simulink model "arducopter"  (R2021a)
settings: Solver=FixedStepAuto  StartTime=0.0  StopTime=simIn.param.timeEnd  FixedStep=simIn.param.dt  RelTol=1e-3
undefined symbols (not defined in the file or in its folder): DiscIntNeverNeededParam, sim, simIn
libraries: simulink x35, slident x4, vrlib x1
(part 4 of 9)

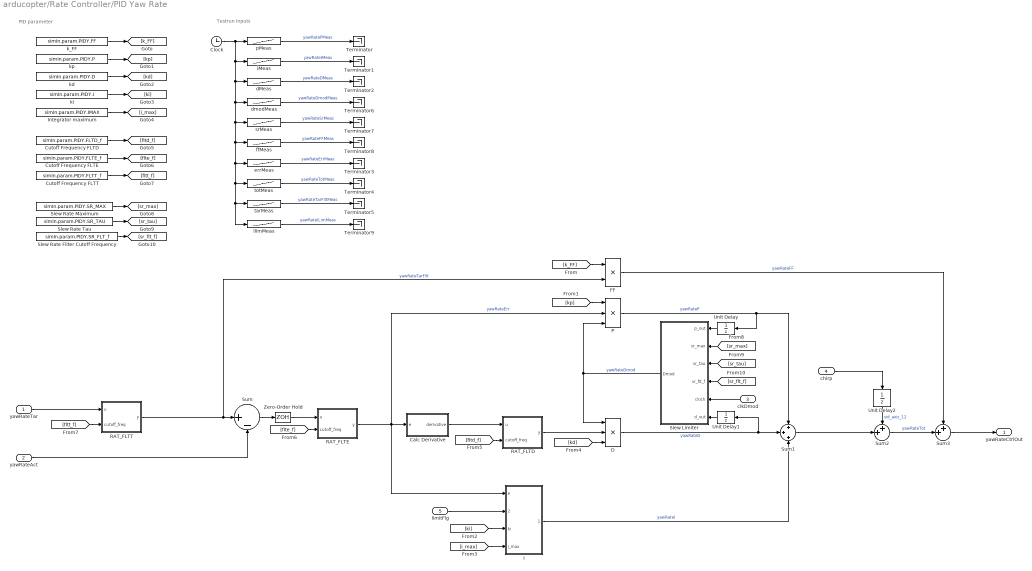
== system arducopter/Rate Controller/PID Yaw Rate ==
  note: PID parameter
  note: Testrun inputs
  yawRateTar : Inport
  yawRateAct : Inport  Port=2
  clkDmod : Inport  Port=3
  chirp : Inport  Port=4
  limitFlg : Inport  Port=5
  Calc Derivative : Subsystem
  Clock : Clock
  Cutoff Frequency FLTD : Constant  Value=simIn.param.PIDY.FLTD_f
  Cutoff Frequency FLTE : Constant  Value=simIn.param.PIDY.FLTE_f
  Cutoff Frequency FLTT : Constant  Value=simIn.param.PIDY.FLTT_f
  D : Product  Inputs=3
  FF : Product
  I : Subsystem
  Integrator maximum : Constant  Value=simIn.param.PIDY.IMAX
  P : Product  Inputs=3
  RAT_FLTD : Subsystem  TreatAsAtomicUnit=on  SystemSampleTime=simIn.param.dt
  RAT_FLTE : Subsystem  TreatAsAtomicUnit=on  SystemSampleTime=simIn.param.dt
  RAT_FLTT : Subsystem  TreatAsAtomicUnit=on  SystemSampleTime=simIn.param.dt
  Slew Limiter : Subsystem
  Slew Rate Filter Cutoff Frequency : Constant  Value=simIn.param.PIDY.SR_FLT_f
  Slew Rate Maximum : Constant  Value=simIn.param.PIDY.SR_MAX
  Slew Rate Tau : Constant  Value=simIn.param.PIDY.SR_TAU
  Sum : Sum  Inputs=|+-
  Sum1 : Sum  Inputs=+|+|+
  Sum2 : Sum  Inputs=++|
  Sum3 : Sum  Inputs=++|  OutDataTypeStr=single
  Terminator{,1..9} (10 alike) : Terminator
  Unit Delay : UnitDelay  InitialCondition=simIn.init.PIDY.P  SampleTime=-1  HasFrameUpgradeWarning=on
  Unit Delay1 : UnitDelay  InitialCondition=simIn.init.PIDY.D  SampleTime=-1  HasFrameUpgradeWarning=on
  Unit Delay2 : UnitDelay  SampleTime=-1  HasFrameUpgradeWarning=on
  Zero-Order Hold : ZeroOrderHold  SampleTime=-1
  dMeas : Lookup_n-D  NumberOfTableDimensions=1  BreakpointsForDimension1=simIn.signals.PIDY.Time  Table=simIn.signals.PIDY.D  InternalRulePriority=Speed  RndMeth=Simplest  InputSameDT=on
  dmodMeas : Lookup_n-D  NumberOfTableDimensions=1  BreakpointsForDimension1=simIn.signals.PIDY.Time  Table=simIn.signals.PIDY.DMod  InternalRulePriority=Speed  RndMeth=Simplest  InputSameDT=on
  errMeas : Lookup_n-D  NumberOfTableDimensions=1  BreakpointsForDimension1=simIn.signals.PIDY.Time  Table=simIn.signals.PIDY.Err  InternalRulePriority=Speed  RndMeth=Simplest  InputSameDT=on
  ffMeas : Lookup_n-D  NumberOfTableDimensions=1  BreakpointsForDimension1=simIn.signals.PIDY.Time  Table=simIn.signals.PIDY.FF  InternalRulePriority=Speed  RndMeth=Simplest  InputSameDT=on
  iMeas : Lookup_n-D  NumberOfTableDimensions=1  BreakpointsForDimension1=simIn.signals.PIDY.Time  Table=simIn.signals.PIDY.I  InternalRulePriority=Speed  RndMeth=Simplest  InputSameDT=on
  ilimMeas : Lookup_n-D  NumberOfTableDimensions=1  BreakpointsForDimension1=simIn.signals.PIDY.Time  Table=simIn.signals.PIDY.ILimit  InternalRulePriority=Speed  RndMeth=Simplest  InputSameDT=on
  k_FF : Constant  Value=simIn.param.PIDY.FF
  kd : Constant  Value=simIn.param.PIDY.D
  ki : Constant  Value=simIn.param.PIDY.I
  kp : Constant  Value=simIn.param.PIDY.P
  pMeas : Lookup_n-D  NumberOfTableDimensions=1  BreakpointsForDimension1=simIn.signals.PIDY.Time  Table=simIn.signals.PIDY.P  InternalRulePriority=Speed  RndMeth=Simplest  InputSameDT=on
  srMeas : Lookup_n-D  NumberOfTableDimensions=1  BreakpointsForDimension1=simIn.signals.PIDY.Time  Table=simIn.signals.PIDY.SRate  InternalRulePriority=Speed  RndMeth=Simplest  InputSameDT=on
  tarMeas : Lookup_n-D  NumberOfTableDimensions=1  BreakpointsForDimension1=simIn.signals.PIDY.Time  Table=simIn.signals.PIDY.Tar  InternalRulePriority=Speed  RndMeth=Simplest  InputSameDT=on
  totMeas : Lookup_n-D  NumberOfTableDimensions=1  BreakpointsForDimension1=simIn.signals.RATE.Time  Table=simIn.signals.RATE.YOut  InternalRulePriority=Speed  RndMeth=Simplest  InputSameDT=on
  yawRateCtrlOut : Outport
  wires:
  RAT_FLTD/1(y) -> D/2
  Sum1/1 -> Sum2/2
  RAT_FLTE/1(y) -> P/2, Calc Derivative/1(e), I/1(e)  "yawRateErr"
  limitFlg/1 -> I/2(limit_flg)
  P/1 -> Unit Delay/1, Sum1/1  "yawRateP"
  Calc Derivative/1(derivative) -> RAT_FLTD/1(u)
  Sum/1 -> Zero-Order Hold/1
  D/1 -> Unit Delay1/1, Sum1/2  "yawRateD"
  I/1(integrator) -> Sum1/3  "yawRateI"
  FF/1 -> Sum3/1  "yawRateFF"
  Sum2/1 -> Sum3/2  "yawRateTot"
  Sum3/1 -> yawRateCtrlOut/1
  RAT_FLTT/1(y) -> FF/2, Sum/1  "yawRateTarFilt"
  yawRateTar/1 -> RAT_FLTT/1(u)
  yawRateAct/1 -> Sum/2
  Zero-Order Hold/1 -> RAT_FLTE/1(u)
  k_FF/1 -> [k_FF]
  kp/1 -> [kp]
  kd/1 -> [kd]
  ki/1 -> [ki]
  Integrator maximum/1 -> [i_max]
  Cutoff Frequency FLTD/1 -> [fltd_f]
  Cutoff Frequency FLTE/1 -> [flte_f]
  Cutoff Frequency FLTT/1 -> [fltt_f]
  [k_FF] -> FF/1
  [kp] -> P/1
  [ki] -> I/3(ki)
  [i_max] -> I/4(i_max)
  [kd] -> D/3
  [fltd_f] -> RAT_FLTD/2(cutoff_freq)
  [flte_f] -> RAT_FLTE/2(cutoff_freq)
  [fltt_f] -> RAT_FLTT/2(cutoff_freq)
  pMeas/1 -> Terminator/1  "yawRatePMeas"
  iMeas/1 -> Terminator1/1  "yawRateIMeas"
  dMeas/1 -> Terminator2/1  "yawRateDMeas"
  totMeas/1 -> Terminator4/1  "yawRateTotMeas"
  tarMeas/1 -> Terminator5/1  "yawRateTarFiltMeas"
  errMeas/1 -> Terminator3/1  "yawRateErrMeas"
  Unit Delay2/1 -> Sum2/1  "sid_axis_12"
  Slew Rate Filter Cutoff Frequency/1 -> [sr_flt_f]
  Slew Rate Maximum/1 -> [sr_max]
  Slew Rate Tau/1 -> [sr_tau]
  dmodMeas/1 -> Terminator6/1  "yawRateDmodMeas"
  srMeas/1 -> Terminator7/1  "yawRateSrMeas"
  ffMeas/1 -> Terminator8/1  "yawRateFFMeas"
  Slew Limiter/1(Dmod) -> D/1, P/3  "yawRateDmod"
  Unit Delay/1 -> Slew Limiter/1(p_out)
  Unit Delay1/1 -> Slew Limiter/6(d_out)
  [sr_max] -> Slew Limiter/2(sr_max)
  [sr_tau] -> Slew Limiter/3(sr_tau)
  [sr_flt_f] -> Slew Limiter/4(sr_flt_f)
  ilimMeas/1 -> Terminator9/1  "yawRateILimMeas"
  clkDmod/1 -> Slew Limiter/5(clock)
  chirp/1 -> Unit Delay2/1
  Clock/1 -> ilimMeas/1, tarMeas/1, totMeas/1, errMeas/1, ffMeas/1, srMeas/1, dmodMeas/1, dMeas/1, iMeas/1, pMeas/1

== system arducopter/Throttle/Input Handler ==
  note: Input Handler
      | Determines source of the inputs to the subsystem, which can
      | be either the real flight data or simulated data.
  inMeas : Inport
  inSim : Inport  Port=2
  thrMan : Inport  Port=3
  Bus Creator : BusCreator  Inputs=9
  Bus Selector : BusSelector  OutputSignals=throttle.thrIn
  Bus Selector1 : BusSelector  OutputSignals=CTUN.thrInMeas,CTUN.angBst,BAT.batRestVoltEst,BAT.batCurr,BAT.batRes,BAT.batVolt,BARO.baroAlt,BARO.baroAirPress,BARO.baroGndTemp
  Switch : Switch  Criteria=u2 > Threshold
  data_in : Outport
  wires:
  inSim/1 -> Bus Selector/1
  inMeas/1 -> Bus Selector1/1
  thrMan/1 -> Switch/2
  Bus Selector/1 -> Switch/3  "<thrIn>"
  Bus Selector1/1 -> Switch/1  "<thrInMeas>"
  Bus Selector1/9 -> Bus Creator/9  "<baroGndTemp>"
  Bus Selector1/8 -> Bus Creator/8  "<baroAirPress>"
  Bus Selector1/7 -> Bus Creator/7  "<baroAlt>"
  Bus Selector1/6 -> Bus Creator/6  "<batVolt>"
  Bus Selector1/5 -> Bus Creator/5  "<batRes>"
  Bus Selector1/4 -> Bus Creator/4  "<batCurr>"
  Bus Selector1/3 -> Bus Creator/3  "<batRestVoltEst>"
  Bus Selector1/2 -> Bus Creator/2  "<angBst>"
  Switch/1 -> Bus Creator/1  "thrTar"
  Bus Creator/1 -> data_in/1

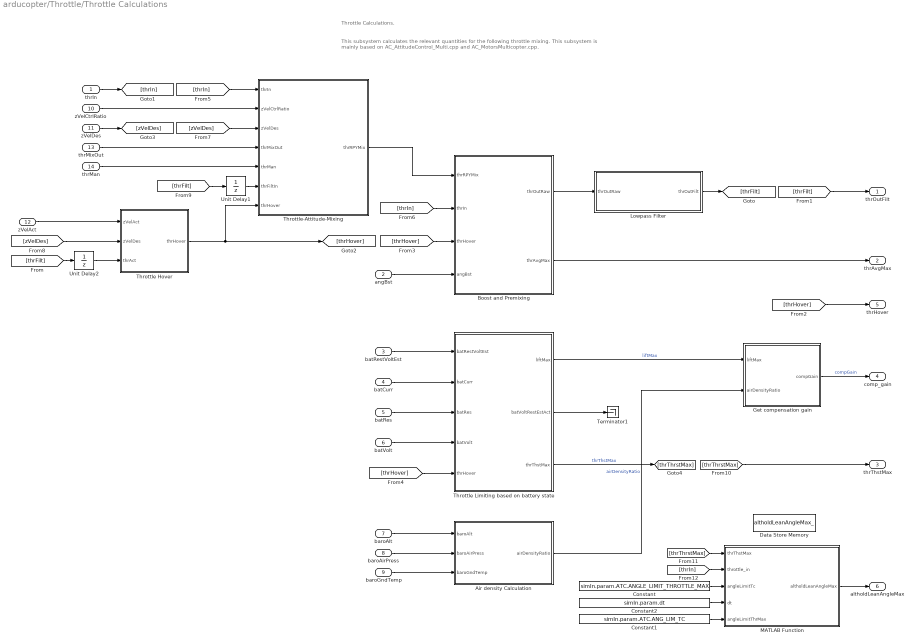
== system arducopter/Throttle/Throttle Calculations ==
  note: Throttle Calculations.
  note: This subsystem calculates the relevant quantities for the following throttle mixing.
      | This subsystem is mainly based on AC_AttitudeControl_Multi.cpp and AC_MotorsMulticopter.cpp.
  thrIn : Inport
  angBst : Inport  Port=2
  batRestVoltEst : Inport  Port=3
  batCurr : Inport  Port=4
  batRes : Inport  Port=5
  batVolt : Inport  Port=6
  baroAlt : Inport  Port=7
  baroAirPress : Inport  Port=8
  baroGndTemp : Inport  Port=9
  zVelCtrlRatio : Inport  Port=10
  zVelDes : Inport  Port=11
  zVelAct : Inport  Port=12
  thrMixOut : Inport  Port=13
  thrMan : Inport  Port=14
  Air density Calculation : Subsystem
  Boost and Premixing : Subsystem  TreatAsAtomicUnit=on  SystemSampleTime=simIn.param.dt
  Constant : Constant  Value=simIn.param.ATC.ANGLE_LIMIT_THROTTLE_MAX
  Constant1 : Constant  Value=simIn.param.ATC.ANG_LIM_TC
  Constant2 : Constant  Value=simIn.param.dt
  Data Store Memory : DataStoreMemory  DataStoreName=altholdLeanAngleMax_  ReadBeforeWriteMsg=warning  WriteAfterWriteMsg=warning  WriteAfterReadMsg=warning  InitialValue=single(0)  ShowAdditionalParam=off  OutDataTypeStr=single
  Get compensation gain : MATLAB Function  TreatAsAtomicUnit=on
  Lowpass Filter : Subsystem
  MATLAB Function : MATLAB Function  TreatAsAtomicUnit=on
  Terminator1 : Terminator
  Throttle Hover : Subsystem  TreatAsAtomicUnit=on  SystemSampleTime=0.1
  Throttle Limiting based on battery state : Subsystem
  Throttle-Attitude-Mixing : Subsystem
  Unit Delay1 : UnitDelay  InitialCondition=simIn.init.CTUN.ThrOut  SampleTime=-1  HasFrameUpgradeWarning=on
  Unit Delay2 : UnitDelay  InitialCondition=simIn.init.CTUN.ThrOut  SampleTime=-1  HasFrameUpgradeWarning=on
  thrOutFilt : Outport
  thrAvgMax : Outport  Port=2
  thrThstMax : Outport  Port=3
  comp_gain : Outport  Port=4
  thrHover : Outport  Port=5
  altholdLeanAngleMax : Outport  Port=6
  wires:
  Throttle Hover/1(thrHover) -> [thrHover], Throttle-Attitude-Mixing/7(thrHover)
  Get compensation gain/1(compGain) -> comp_gain/1  "compGain"
  Throttle Limiting based on battery state/1(liftMax) -> Get compensation gain/1(liftMax)  "liftMax"
  [thrFilt] -> Unit Delay2/1
  Throttle Limiting based on battery state/2(batVoltRestEstAct) -> Terminator1/1
  [thrHover] -> Throttle Limiting based on battery state/5(thrHover)
  Unit Delay2/1 -> Throttle Hover/3(thrAct)
  Throttle Limiting based on battery state/3(thrThstMax) -> [thrThrstMax]  "thrThstMax"
  [thrFilt] -> thrOutFilt/1
  Lowpass Filter/1(thrOutFilt) -> [thrFilt]
  angBst/1 -> Boost and Premixing/4(angBst)
  [thrHover] -> Boost and Premixing/3(thrHover)
  Boost and Premixing/2(thrAvgMax) -> thrAvgMax/1
  batRestVoltEst/1 -> Throttle Limiting based on battery state/1(batRestVoltEst)
  batCurr/1 -> Throttle Limiting based on battery state/2(batCurr)
  batRes/1 -> Throttle Limiting based on battery state/3(batRes)
  batVolt/1 -> Throttle Limiting based on battery state/4(batVolt)
  baroAlt/1 -> Air density Calculation/1(baroAlt)
  baroAirPress/1 -> Air density Calculation/2(baroAirPress)
  baroGndTemp/1 -> Air density Calculation/3(baroGndTemp)
  Boost and Premixing/1(thrOutRaw) -> Lowpass Filter/1(thrOutRaw)
  [thrHover] -> thrHover/1
  [thrIn] -> Boost and Premixing/2(thrIn)
  thrIn/1 -> [thrIn]
  zVelCtrlRatio/1 -> Throttle-Attitude-Mixing/2(zVelCtrlRatio)
  thrMan/1 -> Throttle-Attitude-Mixing/5(thrMan)
  Throttle-Attitude-Mixing/1(thrRPYMix) -> Boost and Premixing/1(thrRPYMix)
  [thrIn] -> Throttle-Attitude-Mixing/1(thrIn)
  zVelDes/1 -> [zVelDes]
  [zVelDes] -> Throttle-Attitude-Mixing/3(zVelDes)
  [zVelDes] -> Throttle Hover/2(zVelDes)
  zVelAct/1 -> Throttle Hover/1(zVelAct)
  Air density Calculation/1(airDensityRatio) -> Get compensation gain/2(airDensityRatio)  "airDensityRatio"
  thrMixOut/1 -> Throttle-Attitude-Mixing/4(thrMixOut)
  [thrFilt] -> Unit Delay1/1
  Unit Delay1/1 -> Throttle-Attitude-Mixing/6(thrFiltIn)
  [thrThrstMax] -> thrThstMax/1
  [thrThrstMax] -> MATLAB Function/1(thrThstMax)
  [thrIn] -> MATLAB Function/2(throttle_in)
  Constant/1 -> MATLAB Function/3(angleLimitTc)
  Constant1/1 -> MATLAB Function/5(angleLimitThrMax)
  Constant2/1 -> MATLAB Function/4(dt)
  MATLAB Function/1(altholdLeanAngleMax) -> altholdLeanAngleMax/1

== system arducopter/Attitude Controller/input_euler_angle_roll_pitch_euler_rate_yaw()/Add feedforward to angVelBody ==
  note: Thrust error angle above which yaw corrections are limited
  angVelBodyFeedforward : Inport
  angVelBodyIn : Inport  Port=2
  thurstErrorAngle : Inport  Port=3
  yawRateAct : Inport  Port=4
  Constant : Constant  Value=simIn.param.ATC.THRUST_ERROR_ANGLE
  MATLAB Function : MATLAB Function  TreatAsAtomicUnit=on
  angVelBody : Outport
  feedforwardScaler : Outport  Port=2
  wires:
  angVelBodyFeedforward/1 -> MATLAB Function/1(angVelBodyFeedforward)
  angVelBodyIn/1 -> MATLAB Function/2(angVelBodyIn)
  thurstErrorAngle/1 -> MATLAB Function/3(thrustErrorAngle)
  yawRateAct/1 -> MATLAB Function/4(yawRateAct)
  MATLAB Function/1(angVelBodyNew) -> angVelBody/1
  Constant/1 -> MATLAB Function/5(maxThrustErrorAngle4YawCorr)
  MATLAB Function/2(feedforwardScaler) -> feedforwardScaler/1

== system arducopter/Attitude Controller/input_euler_angle_roll_pitch_euler_rate_yaw()/Feedforward disabled ==
  note: QuaternionT<T>::from_euler()
      | Computes the quaternion from the given euler angles
  note: This subsystem represents to part of input_euler_angle_roll_pitch_euler_rate_yaw() that is executed, when the feedforward is disabled ( ATC_RATE_FF_ENAB = 0 )
  eulerAngleTar : Inport
  eulerInputDes : Inport  Port=2
  Constant : Constant  Value=0  OutDataTypeStr=single
  Constant1 : Constant  Value=0  OutDataTypeStr=single
  Demux : Demux  Outputs=3
  Gain : Gain  Gain=simIn.param.dt
  MATLAB Function : MATLAB Function  TreatAsAtomicUnit=on
  Selector : Selector  InputPortWidth=3  IndexOptions=Index vector (dialog)  Indices=[3]  OutputSizes=1
  Sum : Sum  Inputs=|++
  eulerRateTar : Outport
  angVelTar : Outport  Port=2
  attitudeTarget : Outport  Port=3
  wires:
  MATLAB Function/1(q) -> attitudeTarget/1  "attitudeTarget"
  Demux/1 -> MATLAB Function/1(roll)
  Demux/2 -> MATLAB Function/2(pitch)
  eulerInputDes/1 -> Demux/1
  Demux/3 -> Gain/1
  Gain/1 -> Sum/1
  Sum/1 -> MATLAB Function/3(yaw)
  eulerAngleTar/1 -> Selector/1
  Constant/1 -> eulerRateTar/1
  Constant1/1 -> angVelTar/1
  Selector/1 -> Sum/2

== system arducopter/Attitude Controller/input_euler_angle_roll_pitch_euler_rate_yaw()/Feedforward enabled ==
  note: euler_rate_to_ang_vel()
      | Converts the target euler rates into a target frame angular velocity vector for feedforward
  note: euler_accel_limit()
      | Translation of acceleration limits eulerAccelMax to the body frame
  note: This subsystem represents to part of input_euler_angle_roll_pitch_euler_rate_yaw() that is executed, when the feedforward is enabled (ATC_RATE_FF_ENAB = 1)
  note: Maximum angular accelerations in earth frame
  note: Input shaping
      | Computes target euler rates based on the error between latest angle target and the desired angle by the pilot, thereby considering acceleration limits.
  note: ang_vel_limit()
      | Ensures that angular velocites do not go over configured rate limits
  note: ang_vel_to_euler_rate()
      | Converts the target body-frame angular velocites into target euler rates
  eulerRateTarIn : Inport
  eulerAngleTar : Inport  Port=2
  eulerInputDes : Inport  Port=3
  Constant : Constant  Value=simIn.param.ATC.ACCEL_R_MAX
  Constant1 : Constant  Value=simIn.param.ATC.ACCEL_P_MAX
  Constant2 : Constant  Value=simIn.param.ATC.ACCEL_Y_MAX
  Constant3 : Constant  Value=simIn.param.ATC.RATE_R_MAX
  Constant4 : Constant  Value=simIn.param.ATC.RATE_P_MAX
  Constant5 : Constant  Value=simIn.param.ATC.RATE_Y_MAX
  Gain : Gain  Gain=pi/180
  Gain1 : Gain  Gain=pi/180
  Gain2 : Gain  Gain=pi/180
  MATLAB Function : MATLAB Function  TreatAsAtomicUnit=on
  MATLAB Function1 : MATLAB Function  TreatAsAtomicUnit=on
  MATLAB Function2 : MATLAB Function  TreatAsAtomicUnit=on
  MATLAB Function3 : MATLAB Function  TreatAsAtomicUnit=on
  Mux : Mux  Inputs=3
  cdeg/ss to rad/ss : Gain  Gain=0.01*pi/180
  input shaping : Subsystem
  eulerRateTarOut : Outport
  angVelTar : Outport  Port=2
  wires:
  [eulerAngleTar] -> MATLAB Function/1(eulerAngleTar), MATLAB Function1/1(eulerAngle), input shaping/1(eulerAngleTar)
  Constant/1 -> Mux/1
  Mux/1 -> cdeg/ss to rad/ss/1
  Constant1/1 -> Mux/2
  Constant2/1 -> Mux/3
  MATLAB Function/1(eulerAccelMaxBF) -> input shaping/4(eulerAccelMax)
  eulerInputDes/1 -> input shaping/2(eulerInputDes)
  eulerRateTarIn/1 -> input shaping/3(eulerRateTarIn)
  input shaping/1(eulerRateTar) -> MATLAB Function1/2(eulerRate)  "eulerRateTar"
  MATLAB Function1/1(angVelTar) -> MATLAB Function2/1(angVelTar)  "angVelTar"
  Gain/1 -> MATLAB Function2/2(angVelRollMax)
  Constant3/1 -> Gain/1
  Constant4/1 -> Gain1/1
  Gain1/1 -> MATLAB Function2/3(angVelPitchMax)
  Gain2/1 -> MATLAB Function2/4(angVelYawMax)
  Constant5/1 -> Gain2/1
  eulerAngleTar/1 -> [eulerAngleTar]  "eulerAngleTar"
  [eulerAngleTar] -> MATLAB Function3/2(eulerAngle)
  MATLAB Function3/1(eulerRate) -> eulerRateTarOut/1
  MATLAB Function2/1(angVelTarLimited) -> [angVelTar]
  [angVelTar] -> MATLAB Function3/1(angVelBf)
  [angVelTar] -> angVelTar/1
  cdeg/ss to rad/ss/1 -> MATLAB Function/2(eulerAccelMaxEF)

== system arducopter/Attitude Controller/input_euler_angle_roll_pitch_euler_rate_yaw()/Update attitudeTarget ==
  note: Normalize attitudeTarget
  note: Use angVelTar to rotate attitudeTarget
  note: Use rotated attitudeTarget, if FF is enabled.
      | Otherwise, use unchanged attitudeTarget
  attitudeTarget : Inport
  angVelTar : Inport  Port=2
  ffEnabled : Inport  Port=3
  MATLAB Function : MATLAB Function  TreatAsAtomicUnit=on
  Rotate target attitude : Subsystem
  Switch : Switch  Criteria=u2 > Threshold
  attitudeTargetUpdate : Outport
  wires:
  MATLAB Function/1(qNorm) -> attitudeTargetUpdate/1
  Switch/1 -> MATLAB Function/1(q)
  ffEnabled/1 -> Switch/2
  attitudeTarget/1 -> Switch/3, Rotate target attitude/1(attitudeTarget)
  angVelTar/1 -> Rotate target attitude/2(angVelTar)
  Rotate target attitude/1(attitudeTargetRot) -> Switch/1

== system arducopter/Attitude Controller/input_euler_angle_roll_pitch_euler_rate_yaw()/reset yaw targets ==
  note: "ahrs.yaw - euler_angle_target.z"
  note: This subsystem resets the yaw target angle and rate, if the throttle is zero, meaning that the copter is landed. The respective function is AC_AttitudeControl::reset_yaw_target_and_rate() , which is called in ModeStabilize::run() when the copter is armed, but throttle is still zero.
  eulerRateTarIn : Inport
  attitudeTargetIn : Inport  Port=2
  eulerAngleAct : Inport  Port=3
  throttle : Inport  Port=4
  Demux : Demux  Outputs=3
  Demux1 : Demux  Outputs=3
  MATLAB Function1 : MATLAB Function  TreatAsAtomicUnit=on
  MATLAB Function5 : MATLAB Function  TreatAsAtomicUnit=on
  MATLAB Function9 : MATLAB Function  TreatAsAtomicUnit=on
  Mux : Mux  Inputs=3
  Mux1 : Mux  Inputs=3
  Subtract : Sum  Inputs=-+
  Switch : Switch  Criteria=u2 > Threshold
  Switch1 : Switch  Criteria=u2 > Threshold
  Terminator{,1..4} (5 alike) : Terminator
  Zero : Constant  Value=0  OutDataTypeStr=single
  Zero1 : Constant  Value=0  OutDataTypeStr=single
  Zero2 : Constant  Value=0  OutDataTypeStr=single
  eulerRateTar : Outport
  attitudeTarget : Outport  Port=2
  wires:
  Switch1/1 -> attitudeTarget/1
  Switch/1 -> eulerRateTar/1
  throttle/1 -> Switch1/2, Switch/2
  eulerRateTarIn/1 -> Demux1/1, Switch/1
  eulerAngleAct/1 -> Demux/1
  MATLAB Function9/1(qRes) -> Switch1/3
  attitudeTargetIn/1 -> Switch1/1, MATLAB Function9/2(q2), MATLAB Function1/1(q)
  MATLAB Function1/3(yaw) -> Subtract/1  "yawAngleTar"
  MATLAB Function1/1(roll) -> Terminator/1
  MATLAB Function1/2(pitch) -> Terminator1/1
  Demux/1 -> Terminator2/1
  Demux/2 -> Terminator3/1
  Demux/3 -> Subtract/2
  Subtract/1 -> Mux/3
  MATLAB Function5/1(q) -> MATLAB Function9/1(q1)  "attitudeTargetUpdate"
  Mux/1 -> MATLAB Function5/1(vec)
  Zero/1 -> Mux/1
  Zero1/1 -> Mux/2
  Mux1/1 -> Switch/3
  Demux1/1 -> Mux1/1
  Demux1/2 -> Mux1/2
  Demux1/3 -> Terminator4/1
  Zero2/1 -> Mux1/3

== system arducopter/Attitude Controller/input_euler_angle_roll_pitch_euler_rate_yaw()/thrust_heading_rotation_angles() ==
  note: Limit yaw error based in maximum acceleration
  note: AC_AttitudeControl::thrust_vector_rotation_angles()
      | Calculation of thrust_angle, thrust_error_angle, attitude_error and thrust_vector_correction
  note: This subsystem contains all the calculations contained in the function AC_AttitudeControl::thrust_heading_rotation_angles() that is called in AC_AttitudeControl::attitude_controller_run_quat()
  attitudeTargetIn : Inport
  attitudeBodyAct : Inport  Port=2
  Yaw error limitation : Subsystem
  thrust_vector_rotation_angles() : Subsystem
  attitudeTarget : Outport
  attitudeError : Outport  Port=2
  thrustErrorAngle : Outport  Port=3
  thrustAngle : Outport  Port=4
  wires:
  attitudeTargetIn/1 -> [attitudeTarget]  "attTar"
  [attitudeBody] -> thrust_vector_rotation_angles()/2(attitudeBodyAct)
  thrust_vector_rotation_angles()/1(attitudeError) -> Yaw error limitation/1(attitudeErrorIn)
  thrust_vector_rotation_angles()/3(thrustErrAngle) -> thrustErrorAngle/1
  thrust_vector_rotation_angles()/2(thrustVecCorrection) -> Yaw error limitation/2(thrustVecCorrection)
  thrust_vector_rotation_angles()/4(thrustAngle) -> thrustAngle/1
  attitudeBodyAct/1 -> [attitudeBody]  "attBody"
  [attitudeBody] -> Yaw error limitation/3(attitudeBody)
  Yaw error limitation/1(atitudeTarget) -> attitudeTarget/1
  Yaw error limitation/2(attitudeError) -> attitudeError/1
  [attitudeTarget] -> thrust_vector_rotation_angles()/1(attitudeTarget)
  [attitudeTarget] -> Yaw error limitation/4(attitudeTarget)

== system arducopter/Attitude Controller/input_euler_angle_roll_pitch_euler_rate_yaw()/update_ang_vel_target_from_att_error() ==
  note: The subsystems either use the square root controller or an easy proportional relation (kp*err) to calculate the target angular velocity
  note: AC_AttitudeControl::update_ang_vel_target_from_att_error()
      | Compute the angular velocity corrections in the body frame from the attitude error.
  attitudeError : Inport
  Calc angular velocity target pitch : Subsystem
  Calc angular velocity target roll : Subsystem
  Calc angular velocity target yaw : Subsystem
  Mux : Mux  Inputs=3
  Selector : Selector  InputPortWidth=3  IndexOptions=Index vector (dialog)  Indices=[1]  OutputSizes=1
  Selector1 : Selector  InputPortWidth=3  IndexOptions=Index vector (dialog)  Indices=[2]  OutputSizes=1
  Selector2 : Selector  InputPortWidth=3  IndexOptions=Index vector (dialog)  Indices=[3]  OutputSizes=1
  angVelBody : Outport
  wires:
  attitudeError/1 -> Selector2/1, Selector/1, Selector1/1
  Mux/1 -> angVelBody/1
  Selector/1 -> Calc angular velocity target roll/1(attitudeErrorRoll)
  Calc angular velocity target roll/1(angVelRoll) -> Mux/1
  Calc angular velocity target yaw/1(angVelYaw) -> Mux/3
  Calc angular velocity target pitch/1(angVelPitch) -> Mux/2
  Selector1/1 -> Calc angular velocity target pitch/1(attitudeErrorPitch)
  Selector2/1 -> Calc angular velocity target yaw/1(attitudeErrorYaw)

== system arducopter/Position Controller/P Position z/Scale Factor Z ==
  note: AP_AHRS::getControlScaleZ()
      | This subsystem calculates a scaling factor for the target of vertical motion quantities based on the EKF type that is being used.
      | Taken from AP_AHRS::getControlScaleZ() in AP_AHRS.cpp. Called in AC_PosControl::update_z_controller().
      | Flying with only DCM lower the gain of the controllers by 4x to cope with high lag.
  ekfType : Inport
  EKF used : Constant  OutDataTypeStr=single
  No EKF : Constant  Value=0.25  OutDataTypeStr=single
  Switch : Switch  Criteria=u2 > Threshold
  scale_z : Outport
  wires:
  ekfType/1 -> Switch/2
  EKF used/1 -> Switch/1
  No EKF/1 -> Switch/3
  Switch/1 -> scale_z/1

== system arducopter/Position Controller/P Position z/Set vertical speed & acceleration limit ==
  note: Calculation of vertical speed and acceleration limits
      | This subsystem corresponds to the function set_correction_speed_accel_z() , in AC_PosControl.cpp,
      | which is called in the ModeLoiter::init() function of mode_loiter.cpp.
      | The intention of this function is to calculate z position error limits, which corresponds to the vertical speed
      | and acceleration limits given by parameters, so that the speed and acceleration limits are still kept after
      | the square root controller was executed without explicitly enforce the limits to the quantities.
  outMin : Inport
  outMax : Inport  Port=2
  DoutMax : Inport  Port=3
  D2OutMax : Inport  Port=4
  kp : Inport  Port=5
  Abs : Abs
  Gain : Gain  Gain=-1
  Inverse Square Root Controller : Subsystem  TreatAsAtomicUnit=on
  Set error limits : MATLAB Function  TreatAsAtomicUnit=on
  errMin : Outport
  errMax : Outport  Port=2
  D1max : Outport  Port=3
  wires:
  Abs/1 -> Gain/1
  Gain/1 -> Set error limits/1(outMin)
  outMax/1 -> Set error limits/2(outMax)
  outMin/1 -> Abs/1
  DoutMax/1 -> Set error limits/3(DoutMax)
  Set error limits/1(errMin) -> errMin/1
  Set error limits/3(D1max) -> D1max/1
  Set error limits/2(errMax) -> errMax/1
  D2OutMax/1 -> Set error limits/4(D2OutMax)
  kp/1 -> Set error limits/5(kp)

== system arducopter/Position Controller/PID Acceleration z/Calc Derivative ==
  e : Inport
  ATC input time constant : Constant  Value=simIn.param.dt
  Divide : Product  Inputs=*/
  Sum : Sum  Inputs=|+-
  Unit Delay : UnitDelay  SampleTime=-1  HasFrameUpgradeWarning=on
  derivative : Outport
  wires:
  e/1 -> Sum/1, Unit Delay/1
  Unit Delay/1 -> Sum/2
  Sum/1 -> Divide/1
  ATC input time constant/1 -> Divide/2
  Divide/1 -> derivative/1

== system arducopter/Position Controller/PID Acceleration z/I ==
  note: Integrator, see AC_PID.cpp, line 230
      | Initialization: set_integrator() in AC_PosControl::init_z_controller()
  e : Inport
  limitFlg : Inport  Port=2
  ki : Inport  Port=3
  i_max : Inport  Port=4
  Constant1 : Constant  Value=simIn.param.dt
  Data Type Conversion1 : DataTypeConversion  OutDataTypeStr=single
  IC1 : InitialCondition  Value=simIn.init.PIDA.I
  Integrator : MATLAB Function  TreatAsAtomicUnit=on
  Unit Delay1 : UnitDelay  InitialCondition=simIn.init.PIDA.I  SampleTime=-1  HasFrameUpgradeWarning=on
  integrator : Outport
  wires:
  e/1 -> Integrator/1(error)
  Integrator/1(integrator_out) -> IC1/1
  [integrator_out] -> integrator/1
  Constant1/1 -> Data Type Conversion1/1
  limitFlg/1 -> Integrator/3(limit_flg)
  [integrator_out] -> Unit Delay1/1
  IC1/1 -> [integrator_out]
  Unit Delay1/1 -> Integrator/2(integrator)
  ki/1 -> Integrator/4(ki)
  i_max/1 -> Integrator/5(i_max)
  Data Type Conversion1/1 -> Integrator/6(dt)

== system arducopter/Position Controller/PID Acceleration z/RAT_FLTD ==
  note: Digital Filter:
      | $y_n = (1 - \alpha)y_{n-1} + x \cdot \alpha$
  note: Alpha Calculation:
      | $\alpha = \frac{\mathrm{d}t}{\mathrm{d}t + 2 \pi f_{\mathrm{Cutoff}}$
  note: See AC_PID.cpp, line 144.
  note: See AP_Math.cpp, line 393.
  u : Inport
  cutoff_freq : Inport  Port=2
  ATC input time constant : Constant  Value=simIn.param.dt
  Add : Sum
  Calculate Alpha : Product  Inputs=*/
  Compare To Zero : simulink/Logic and Bit Operations/Compare To Zero  relop=<=  OutDataTypeStr=boolean
  Compare To Zero1 : simulink/Logic and Bit Operations/Compare To Zero  relop=<=  OutDataTypeStr=boolean
  Constant2 : Constant  OutDataTypeStr=single
  Constant3 : Constant  OutDataTypeStr=single
  Constant4 : Constant  OutDataTypeStr=single
  Data Type Conversion1 : DataTypeConversion  OutDataTypeStr=single
  Divide : Product  Inputs=*/
  Gain : Gain  Gain=2*pi
  IC : InitialCondition  Value=simIn.init.PIDA.DerFilt
  Logical Operator : Logic  Operator=OR  AllPortsSameDT=off  OutDataTypeStr=boolean
  Product : Product
  Product1 : Product
  Subtract1 : Sum  Inputs=+-
  Sum : Sum  Inputs=++|  OutDataTypeStr=single
  Switch : Switch  Criteria=u2 > Threshold
  Unit Delay : UnitDelay  SampleTime=-1  HasFrameUpgradeWarning=on
  y : Outport
  wires:
  Product1/1 -> Sum/2
  Unit Delay/1 -> Product1/2
  Subtract1/1 -> Product1/1
  [alpha] -> Subtract1/2
  Constant2/1 -> Subtract1/1
  [alpha] -> Product/1
  Calculate Alpha/1 -> Switch/3
  Add/1 -> Calculate Alpha/2
  [dt] -> Add/1, Calculate Alpha/1
  Gain/1 -> Divide/2
  cutoff_freq/1 -> [cutoff_freq]
  u/1 -> Product/2
  Divide/1 -> Add/2
  Constant3/1 -> Divide/1
  Product/1 -> Sum/1
  Switch/1 -> [alpha]
  ATC input time constant/1 -> Data Type Conversion1/1
  [cutoff_freq] -> Gain/1
  [dt] -> Compare To Zero/1
  [cutoff_freq] -> Compare To Zero1/1
  Compare To Zero/1 -> Logical Operator/1
  Compare To Zero1/1 -> Logical Operator/2
  Logical Operator/1 -> Switch/2
  Constant4/1 -> Switch/1
  Sum/1 -> IC/1
  IC/1 -> Unit Delay/1, y/1
  Data Type Conversion1/1 -> [dt]

== system arducopter/Position Controller/PID Acceleration z/RAT_FLTE ==
  note: Digital Filter:
      | $y_n = (1 - \alpha)y_{n-1} + x \cdot \alpha$
  note: Alpha Calculation:
      | $\alpha = \frac{\mathrm{d}t}{\mathrm{d}t + 2 \pi f_{\mathrm{Cutoff}}$
  note: See AC_PID.cpp, line 144.
  note: See AP_Math.cpp, line 393.
  u : Inport
  cutoff_freq : Inport  Port=2
  ATC input time constant : Constant  Value=simIn.param.dt
  Add : Sum
  Calculate Alpha : Product  Inputs=*/
  Compare To Zero : simulink/Logic and Bit Operations/Compare To Zero  relop=<=  OutDataTypeStr=boolean
  Compare To Zero1 : simulink/Logic and Bit Operations/Compare To Zero  relop=<=  OutDataTypeStr=boolean
  Constant2 : Constant  OutDataTypeStr=single
  Constant3 : Constant  OutDataTypeStr=single
  Constant4 : Constant  OutDataTypeStr=single
  Data Type Conversion1 : DataTypeConversion  OutDataTypeStr=single
  Divide : Product  Inputs=*/
  Gain : Gain  Gain=2*pi
  IC : InitialCondition  Value=simIn.init.PIDA.ErrFilt
  Logical Operator : Logic  Operator=OR  AllPortsSameDT=off  OutDataTypeStr=boolean
  Product : Product
  Product1 : Product
  Subtract1 : Sum  Inputs=+-
  Sum : Sum  Inputs=++|  OutDataTypeStr=single
  Switch : Switch  Criteria=u2 > Threshold
  Unit Delay : UnitDelay  SampleTime=-1  HasFrameUpgradeWarning=on
  y : Outport
  wires:
  Product1/1 -> Sum/2
  Unit Delay/1 -> Product1/2
  Subtract1/1 -> Product1/1
  [alpha] -> Subtract1/2
  Constant2/1 -> Subtract1/1
  [alpha] -> Product/1
  Calculate Alpha/1 -> Switch/3
  Add/1 -> Calculate Alpha/2
  [dt] -> Add/1, Calculate Alpha/1
  Gain/1 -> Divide/2
  cutoff_freq/1 -> [cutoff_freq]
  u/1 -> Product/2
  Divide/1 -> Add/2
  Constant3/1 -> Divide/1
  Product/1 -> Sum/1
  Switch/1 -> [alpha]
  ATC input time constant/1 -> Data Type Conversion1/1
  [cutoff_freq] -> Gain/1
  [dt] -> Compare To Zero/1
  [cutoff_freq] -> Compare To Zero1/1
  Compare To Zero/1 -> Logical Operator/1
  Compare To Zero1/1 -> Logical Operator/2
  Logical Operator/1 -> Switch/2
  Constant4/1 -> Switch/1
  Sum/1 -> IC/1
  IC/1 -> Unit Delay/1, y/1
  Data Type Conversion1/1 -> [dt]

== system arducopter/Position Controller/PID Acceleration z/RAT_FLTT ==
  note: See AP_Math.cpp, line 393.
  note: See AC_PID.cpp, line 144.
  note: Alpha Calculation:
      | $\alpha = \frac{\mathrm{d}t}{\mathrm{d}t + 2 \pi f_{\mathrm{Cutoff}}$
  note: Digital Filter:
      | $y_n = (1 - \alpha)y_{n-1} + x \cdot \alpha$
  u : Inport
  cutoff_freq : Inport  Port=2
  ATC input time constant : Constant  Value=simIn.param.dt
  Add : Sum
  Calculate Alpha : Product  Inputs=*/
  Compare To Zero : simulink/Logic and Bit Operations/Compare To Zero  relop=<=  OutDataTypeStr=boolean
  Compare To Zero1 : simulink/Logic and Bit Operations/Compare To Zero  relop=<=  OutDataTypeStr=boolean
  Constant2 : Constant  OutDataTypeStr=single
  Constant3 : Constant  OutDataTypeStr=single
  Constant4 : Constant  OutDataTypeStr=single
  Data Type Conversion1 : DataTypeConversion  OutDataTypeStr=single
  Divide : Product  Inputs=*/
  Gain : Gain  Gain=2*pi
  IC : InitialCondition  Value=simIn.init.PIDA.TarFilt
  Logical Operator : Logic  Operator=OR  AllPortsSameDT=off  OutDataTypeStr=boolean
  Product : Product
  Product1 : Product
  Subtract1 : Sum  Inputs=+-
  Sum : Sum  Inputs=++|
  Switch : Switch  Criteria=u2 > Threshold
  Unit Delay : UnitDelay  SampleTime=-1  HasFrameUpgradeWarning=on
  y : Outport
  wires:
  Constant4/1 -> Switch/1
  Logical Operator/1 -> Switch/2
  Compare To Zero1/1 -> Logical Operator/2
  Compare To Zero/1 -> Logical Operator/1
  [cutoff_freq] -> Compare To Zero1/1
  [dt] -> Compare To Zero/1
  [cutoff_freq] -> Gain/1
  ATC input time constant/1 -> Data Type Conversion1/1
  Switch/1 -> [alpha]
  Product/1 -> Sum/1
  Constant3/1 -> Divide/1
  Divide/1 -> Add/2
  u/1 -> Product/2
  cutoff_freq/1 -> [cutoff_freq]
  Gain/1 -> Divide/2
  [dt] -> Calculate Alpha/1, Add/1
  Add/1 -> Calculate Alpha/2
  Calculate Alpha/1 -> Switch/3
  [alpha] -> Product/1
  Constant2/1 -> Subtract1/1
  [alpha] -> Subtract1/2
  Subtract1/1 -> Product1/1
  Product1/1 -> Sum/2
  Sum/1 -> IC/1
  Unit Delay/1 -> Product1/2
  IC/1 -> y/1, Unit Delay/1
  Data Type Conversion1/1 -> [dt]

== system arducopter/Position Controller/PID Acceleration z/Slew Limiter ==
  note: Data Store Memory Elements: Global variables of subsystem
  note: Slew Limiter
      |
      | Calculates the slew limit modifiert Dmod for the P and D part of the controller. The calculation of Dmod is taken from SlewLimiter::modifier() in SlewLimiter.cpp.
  p_out : Inport
  sr_max : Inport  Port=2
  sr_tau : Inport  Port=3
  sr_flt_f : Inport  Port=4
  clock : Inport  Port=5
  d_out : Inport  Port=6
  ATC sample time1 : Constant  Value=simIn.param.dt
  Calculate Dmod : MATLAB Function  TreatAsAtomicUnit=on
  Constant7 : Constant  Value=simIn.param.LOOP_RATE
  Data Store Memory : DataStoreMemory  DataStoreName=pos_event_stored  ReadBeforeWriteMsg=warning  WriteAfterWriteMsg=warning  WriteAfterReadMsg=warning  InitialValue=false  ShowAdditionalParam=off  OutDataTypeStr=boolean
  Data Store Memory1 : DataStoreMemory  DataStoreName=neg_event_stored  ReadBeforeWriteMsg=warning  WriteAfterWriteMsg=warning  WriteAfterReadMsg=warning  InitialValue=false  ShowAdditionalParam=off  OutDataTypeStr=boolean
  Data Store Memory10 : DataStoreMemory  DataStoreName=modifier_slew_rate  ReadBeforeWriteMsg=warning  WriteAfterWriteMsg=warning  WriteAfterReadMsg=warning  InitialValue=simIn.init.PIDA.SROut  ShowAdditionalParam=off  OutDataTypeStr=single
  Data Store Memory11 : DataStoreMemory  DataStoreName=output_slew_rate  ReadBeforeWriteMsg=warning  WriteAfterWriteMsg=warning  WriteAfterReadMsg=warning  InitialValue=simIn.init.PIDA.SROut  ShowAdditionalParam=off  OutDataTypeStr=single
  Data Store Memory2 : DataStoreMemory  DataStoreName=pos_event_idx  ReadBeforeWriteMsg=warning  WriteAfterWriteMsg=warning  WriteAfterReadMsg=warning  InitialValue=1  ShowAdditionalParam=off  OutDataTypeStr=int8
  Data Store Memory3 : DataStoreMemory  DataStoreName=neg_event_idx  ReadBeforeWriteMsg=warning  WriteAfterWriteMsg=warning  WriteAfterReadMsg=warning  InitialValue=1  ShowAdditionalParam=off  OutDataTypeStr=int8
  Data Store Memory4 : DataStoreMemory  DataStoreName=pos_event_ms  ReadBeforeWriteMsg=warning  WriteAfterWriteMsg=warning  WriteAfterReadMsg=warning  InitialValue=[0 0]  ShowAdditionalParam=off  OutDataTypeStr=uint32  Dimensions=2
  Data Store Memory5 : DataStoreMemory  DataStoreName=neg_event_ms  ReadBeforeWriteMsg=warning  WriteAfterWriteMsg=warning  WriteAfterReadMsg=warning  InitialValue=[0 0]  ShowAdditionalParam=off  OutDataTypeStr=uint32  Dimensions=2
  Data Store Memory6 : DataStoreMemory  DataStoreName=max_pos_slew_rate  ReadBeforeWriteMsg=warning  WriteAfterWriteMsg=warning  WriteAfterReadMsg=warning  ShowAdditionalParam=off  OutDataTypeStr=single
  Data Store Memory7 : DataStoreMemory  DataStoreName=max_pos_slew_event_ms  ReadBeforeWriteMsg=warning  WriteAfterWriteMsg=warning  WriteAfterReadMsg=warning  ShowAdditionalParam=off  OutDataTypeStr=uint32
  Data Store Memory8 : DataStoreMemory  DataStoreName=max_neg_slew_rate  ReadBeforeWriteMsg=warning  WriteAfterWriteMsg=warning  WriteAfterReadMsg=warning  ShowAdditionalParam=off  OutDataTypeStr=single
  Data Store Memory9 : DataStoreMemory  DataStoreName=max_neg_slew_event_ms  ReadBeforeWriteMsg=warning  WriteAfterWriteMsg=warning  WriteAfterReadMsg=warning  ShowAdditionalParam=off  OutDataTypeStr=uint32
  Data Store Read : DataStoreRead  DataStoreName=modifier_slew_rate  DataStoreElements=modifier_slew_rate  IndexOptions=Index vector (dialog)  Indices=1  OutputSizes=1
  Data Store Read1 : DataStoreRead  DataStoreName=output_slew_rate  DataStoreElements=output_slew_rate  IndexOptions=Index vector (dialog)  Indices=1  OutputSizes=1
  Data Type Conversion1 : DataTypeConversion  OutDataTypeStr=single
  IC : InitialCondition  Value=2*simIn.init.PIDA.SROut
  Lowpass Filter : MATLAB Function  TreatAsAtomicUnit=on
  Subsystem : Subsystem
  Terminator : Terminator
  Terminator1 : Terminator
  Unit Delay1 : UnitDelay  SampleTime=-1  HasFrameUpgradeWarning=on
  Dmod : Outport
  wires:
  Constant7/1 -> Lowpass Filter/3(loop_rate)
  sr_flt_f/1 -> Lowpass Filter/2(cutoff_freq)
  Lowpass Filter/1(out) -> IC/1  "zAccSrFilt"
  Unit Delay1/1 -> Lowpass Filter/4(out_last)
  Calculate Dmod/1(Dmod) -> Dmod/1  "zAccDmod"
  sr_max/1 -> Calculate Dmod/2(sr_max)
  sr_tau/1 -> Calculate Dmod/3(sr_tau)
  ATC sample time1/1 -> Data Type Conversion1/1
  Data Store Read/1 -> Terminator/1  "zAccSrMod"
  Data Store Read1/1 -> Terminator1/1  "zAccSrOut"
  p_out/1 -> Subsystem/1(p_out)
  d_out/1 -> Subsystem/2(d_out)
  Subsystem/1(sr_raw) -> Lowpass Filter/1(in)  "zAccSrRaw"
  Data Type Conversion1/1 -> Calculate Dmod/4(dt)
  IC/1 -> Unit Delay1/1, Calculate Dmod/1(slew_rate)
  clock/1 -> Calculate Dmod/5(time)

== system arducopter/Position Controller/PID Acceleration z/i_max check ==
  note: Ensure imax is always large enough to overpower hover throttle
      | Check for sufficient high imax is taken from AC_PosControl.cpp, line 984-986.
  thrHover : Inport
  i_max_ : Inport  Port=2
  Gain : Gain  Gain=1000
  Relational Operator : RelationalOperator  Operator=>  OutDataTypeStr=boolean  RndMeth=Simplest
  Switch : Switch  Criteria=u2 > Threshold
  i_max : Outport
  wires:
  thrHover/1 -> Gain/1
  Gain/1 -> Switch/1, Relational Operator/1
  i_max_/1 -> Switch/3, Relational Operator/2
  Relational Operator/1 -> Switch/2
  Switch/1 -> i_max/1

== system arducopter/Position Controller/PID Velocity z/Calc Derivative ==
  e : Inport
  ATC input time constant : Constant  Value=simIn.param.dt
  Divide : Product  Inputs=*/
  Sum : Sum  Inputs=|+-
  Unit Delay : UnitDelay  SampleTime=-1  HasFrameUpgradeWarning=on
  derivative : Outport
  wires:
  e/1 -> Sum/1, Unit Delay/1
  Unit Delay/1 -> Sum/2
  Sum/1 -> Divide/1
  ATC input time constant/1 -> Divide/2
  Divide/1 -> derivative/1

== system arducopter/Position Controller/PID Velocity z/I ==
  note: Integrator, see AC_PID_Basic::update_i()
      | Initialization: integrator=0 (see AC_PosControl::init_z())
  e : Inport
  limitNeg : Inport  Port=2
  limitPos : Inport  Port=3
  ki : Inport  Port=4
  i_max : Inport  Port=5
  Constant1 : Constant  Value=simIn.param.dt
  Data Type Conversion1 : DataTypeConversion  OutDataTypeStr=single
  IC1 : InitialCondition  Value=0
  Integrator : MATLAB Function  TreatAsAtomicUnit=on
  Unit Delay1 : UnitDelay  InitialCondition=single(0)  SampleTime=-1  HasFrameUpgradeWarning=on
  integrator : Outport
  wires:
  e/1 -> Integrator/1(error)
  Integrator/1(integrator_out) -> IC1/1
  [integrator_out] -> integrator/1
  Constant1/1 -> Data Type Conversion1/1
  limitNeg/1 -> Integrator/3(limitNeg)
  [integrator_out] -> Unit Delay1/1
  IC1/1 -> [integrator_out]
  Unit Delay1/1 -> Integrator/2(integrator)
  ki/1 -> Integrator/5(ki)
  i_max/1 -> Integrator/6(i_max)
  Data Type Conversion1/1 -> Integrator/7(dt)
  limitPos/1 -> Integrator/4(limitPos)

== system arducopter/Position Controller/PID Velocity z/RAT_FLTD ==
  note: Digital Filter:
      | $y_n = (1 - \alpha)y_{n-1} + x \cdot \alpha$
  note: Alpha Calculation:
      | $\alpha = \frac{\mathrm{d}t}{\mathrm{d}t + 2 \pi f_{\mathrm{Cutoff}}$
  note: See AC_PID.cpp, update_all()
  note: See AP_Math.cpp, calc_lowpass_alpha_dt()
  u : Inport
  cutoff_freq : Inport  Port=2
  ATC input time constant : Constant  Value=simIn.param.dt
  Add : Sum
  Calculate Alpha : Product  Inputs=*/
  Compare To Zero : simulink/Logic and Bit Operations/Compare To Zero  relop=<=  OutDataTypeStr=boolean
  Compare To Zero1 : simulink/Logic and Bit Operations/Compare To Zero  relop=<=  OutDataTypeStr=boolean
  Constant2 : Constant  OutDataTypeStr=single
  Constant3 : Constant  OutDataTypeStr=single
  Constant4 : Constant  OutDataTypeStr=single
  Data Type Conversion1 : DataTypeConversion  OutDataTypeStr=single
  Divide : Product  Inputs=*/
  Gain : Gain  Gain=2*pi
  IC : InitialCondition  Value=0
  Logical Operator : Logic  Operator=OR  AllPortsSameDT=off  OutDataTypeStr=boolean
  Product : Product
  Product1 : Product
  Subtract1 : Sum  Inputs=+-
  Sum : Sum  Inputs=++|  OutDataTypeStr=single
  Switch : Switch  Criteria=u2 > Threshold
  Unit Delay : UnitDelay  SampleTime=-1  HasFrameUpgradeWarning=on
  y : Outport
  wires:
  Product1/1 -> Sum/2
  Unit Delay/1 -> Product1/2
  Subtract1/1 -> Product1/1
  [alpha] -> Subtract1/2
  Constant2/1 -> Subtract1/1
  [alpha] -> Product/1
  Calculate Alpha/1 -> Switch/3
  Add/1 -> Calculate Alpha/2
  [dt] -> Add/1, Calculate Alpha/1
  Gain/1 -> Divide/2
  cutoff_freq/1 -> [cutoff_freq]
  u/1 -> Product/2
  Divide/1 -> Add/2
  Constant3/1 -> Divide/1
  Product/1 -> Sum/1
  Switch/1 -> [alpha]
  ATC input time constant/1 -> Data Type Conversion1/1
  [cutoff_freq] -> Gain/1
  [dt] -> Compare To Zero/1
  [cutoff_freq] -> Compare To Zero1/1
  Compare To Zero/1 -> Logical Operator/1
  Compare To Zero1/1 -> Logical Operator/2
  Logical Operator/1 -> Switch/2
  Constant4/1 -> Switch/1
  Sum/1 -> IC/1
  IC/1 -> Unit Delay/1, y/1
  Data Type Conversion1/1 -> [dt]

== system arducopter/Position Controller/PID Velocity z/RAT_FLTE ==
  note: Digital Filter:
      | $y_n = (1 - \alpha)y_{n-1} + x \cdot \alpha$
  note: Alpha Calculation:
      | $\alpha = \frac{\mathrm{d}t}{\mathrm{d}t + 2 \pi f_{\mathrm{Cutoff}}$
  note: See AC_PID.cpp, update_all()
  note: See AP_Math.cpp, calc_lowpass_alpha_dt()
  u : Inport
  cutoff_freq : Inport  Port=2
  ATC input time constant : Constant  Value=simIn.param.dt
  Add : Sum
  Calculate Alpha : Product  Inputs=*/
  Compare To Zero : simulink/Logic and Bit Operations/Compare To Zero  relop=<=  OutDataTypeStr=boolean
  Compare To Zero1 : simulink/Logic and Bit Operations/Compare To Zero  relop=<=  OutDataTypeStr=boolean
  Constant2 : Constant  OutDataTypeStr=single
  Constant3 : Constant  OutDataTypeStr=single
  Constant4 : Constant  OutDataTypeStr=single
  Data Type Conversion1 : DataTypeConversion  OutDataTypeStr=single
  Divide : Product  Inputs=*/
  Gain : Gain  Gain=2*pi
  IC : InitialCondition  Value=0
  Logical Operator : Logic  Operator=OR  AllPortsSameDT=off  OutDataTypeStr=boolean
  Product : Product
  Product1 : Product
  Subtract1 : Sum  Inputs=+-
  Sum : Sum  Inputs=++|  OutDataTypeStr=single
  Switch : Switch  Criteria=u2 > Threshold
  Unit Delay : UnitDelay  SampleTime=-1  HasFrameUpgradeWarning=on
  y : Outport
  wires:
  Product1/1 -> Sum/2
  Unit Delay/1 -> Product1/2
  Subtract1/1 -> Product1/1
  [alpha] -> Subtract1/2
  Constant2/1 -> Subtract1/1
  [alpha] -> Product/1
  Calculate Alpha/1 -> Switch/3
  Add/1 -> Calculate Alpha/2
  [dt] -> Add/1, Calculate Alpha/1
  Gain/1 -> Divide/2
  cutoff_freq/1 -> [cutoff_freq]
  u/1 -> Product/2
  Divide/1 -> Add/2
  Constant3/1 -> Divide/1
  Product/1 -> Sum/1
  Switch/1 -> [alpha]
  ATC input time constant/1 -> Data Type Conversion1/1
  [cutoff_freq] -> Gain/1
  [dt] -> Compare To Zero/1
  [cutoff_freq] -> Compare To Zero1/1
  Compare To Zero/1 -> Logical Operator/1
  Compare To Zero1/1 -> Logical Operator/2
  Logical Operator/1 -> Switch/2
  Constant4/1 -> Switch/1
  Sum/1 -> IC/1
  IC/1 -> Unit Delay/1, y/1
  Data Type Conversion1/1 -> [dt]

== system arducopter/Position Controller/PID Velocity z/Scale Factor Z ==
  note: AP_AHRS::getControlScaleZ()
      | This subsystem calculates a scaling factor for the target of vertical motion quantities based on the EKF type that is being used.
      | Taken from AP_AHRS::getControlScaleZ() in AP_AHRS.cpp. Called in AC_PosControl::update_z_controller().
      | Flying with only DCM lower the gain of the controllers by 4x to cope with high lag.
  ekfType : Inport
  EKF used : Constant  OutDataTypeStr=single
  No EKF : Constant  Value=0.25  OutDataTypeStr=single
  Switch : Switch  Criteria=u2 > Threshold
  scale_z : Outport
  wires:
  ekfType/1 -> Switch/2
  EKF used/1 -> Switch/1
  No EKF/1 -> Switch/3
  Switch/1 -> scale_z/1

== system arducopter/Position Controller/calc des climb rate/constrain climb rate ==
  note: Based on get_pilot_speed_dn()
      | Use maximum up-speed if down-speed limit is 0
  in : Inport
  Abs : Abs
  Abs1 : Abs
  Constant1 : Constant  Value=simIn.param.PSCD.VEL_MAX_DN
  Constant2 : Constant  Value=simIn.param.PSCD.VEL_MAX_UP
  Constant3 : Constant  Value=simIn.param.PSCD.VEL_MAX_UP
  Gain : Gain  Gain=-1
  Saturation Dynamic : simulink/Discontinuities/Saturation Dynamic  OutMin=[]  OutMax=[]  OutDataTypeStr=Inherit: Same as second input  OutDataType=fixdt(1, 16)  OutScaling=2^-10  DoSatur=off
  Switch : Switch  Criteria=u2 > Threshold
  out : Outport
  wires:
  Constant1/1 -> Abs/1, Switch/2
  Constant2/1 -> Abs1/1
  Abs/1 -> Switch/1
  Abs1/1 -> Switch/3
  Saturation Dynamic/1 -> out/1
  Switch/1 -> Gain/1
  Gain/1 -> Saturation Dynamic/3
  in/1 -> Saturation Dynamic/2
  Constant3/1 -> Saturation Dynamic/1

== system arducopter/Position Controller/set_pos_target_z_from_climb_rate()/input_vel_accel_z ==
  note: input_vel_accel_z()
      | This subsystem takes the current target position (posTarIn) and desired velocity and acceleration (velDesTar and accDesTar).
      | First, it updates the target position and desired velocity based on the current desired acceleration (accDesIn) (1).
      | Secondly, it calculates the required jerk limited adjustment to the acceleration for the next time dt (accDes) to reach the desired velocity and acceleration targets (velDesTar and accDesTar) (2).
  note: (2) shape_vel_accel()
      | Adjustment of the desired acceleration to follow a jerk limited kinematic path to vel and acc
  note: (1) update_pos_vel_accel()
      | Adjust desired position and velocity based on desired acceleration
  note: Calculate overspeed gain to calculate increased max accel and jerk if over speed
  velDesTar : Inport
  accDesTar : Inport  Port=2
  limitVectorZ : Inport  Port=3
  velMaxUp : Inport  Port=4
  velMaxDn : Inport  Port=5
  accMaxZ : Inport  Port=6
  jerkMax : Inport  Port=7
  posTarIn : Inport  Port=8
  posErr : Inport  Port=9
  velErr : Inport  Port=10
  velDesIn : Inport  Port=11
  accDesIn : Inport  Port=12
  Constant : Constant  Value=simIn.param.PSCD.OVERSPEED_GAIN_Z
  Constant1 : Constant  OutDataTypeStr=boolean
  Constant2 : Constant  Value=simIn.param.dt  OutDataTypeStr=single
  MATLAB Function : MATLAB Function  TreatAsAtomicUnit=on
  Product : Product
  Product1 : Product
  calc accMin : Subsystem
  shape_vel_accel : Subsystem
  update_pos_vel_accel : Subsystem
  posTar : Outport
  velDes : Outport  Port=2
  accDes : Outport  Port=3
  wires:
  velMaxUp/1 -> MATLAB Function/1(velMaxUp)
  accMaxZ/1 -> Product/2
  velDesIn/1 -> [velDesIn]
  velMaxDn/1 -> MATLAB Function/2(velMaxDn)
  Constant/1 -> MATLAB Function/4(overspeedGainDefault)
  [velDesIn] -> MATLAB Function/3(velDes)
  posTarIn/1 -> update_pos_vel_accel/1(posTarIn)
  [velDesIn] -> update_pos_vel_accel/2(velDesIn)
  accDesIn/1 -> [accDesIn]
  limitVectorZ/1 -> update_pos_vel_accel/4(limitVectorZ)
  update_pos_vel_accel/2(velDes) -> [velDes]
  accDesTar/1 -> shape_vel_accel/2(acc)
  velDesTar/1 -> shape_vel_accel/1(vel)
  [accDesIn] -> update_pos_vel_accel/3(accDesIn)
  [accDesIn] -> shape_vel_accel/4(accDes)
  [accMax] -> calc accMin/1(accMax), shape_vel_accel/6(accMax)
  calc accMin/1(accMin) -> shape_vel_accel/5(accMin)
  Constant2/1 -> shape_vel_accel/8(dt)
  Constant1/1 -> shape_vel_accel/9(limitTotalAccel)
  update_pos_vel_accel/1(posTar) -> posTar/1
  [velDes] -> shape_vel_accel/3(velDes)
  [velDes] -> velDes/1
  shape_vel_accel/1(accDesShaped) -> accDes/1
  MATLAB Function/1(overspeedGain) -> Product1/1, Product/1
  Product/1 -> [accMax]
  jerkMax/1 -> Product1/2
  Product1/1 -> [jerkMax]
  [jerkMax] -> shape_vel_accel/7(jerkMax)
  posErr/1 -> update_pos_vel_accel/5(posErr)
  velErr/1 -> update_pos_vel_accel/6(velErr)

== system arducopter/Rate Controller/PID Pitch Rate/Calc Derivative ==
  e : Inport
  ATC input time constant : Constant  Value=simIn.param.dt
  Data Type Conversion1 : DataTypeConversion  OutDataTypeStr=single
  Divide : Product  Inputs=*/
  Sum : Sum  Inputs=|+-
  Unit Delay : UnitDelay  SampleTime=-1  HasFrameUpgradeWarning=on
  derivative : Outport
  wires:
  Divide/1 -> derivative/1
  ATC input time constant/1 -> Data Type Conversion1/1
  Sum/1 -> Divide/1
  Unit Delay/1 -> Sum/2
  e/1 -> Unit Delay/1, Sum/1
  Data Type Conversion1/1 -> Divide/2

== system arducopter/Rate Controller/PID Pitch Rate/I ==
  note: Integrator, see AC_PID::update_i()
  e : Inport
  limit_flg : Inport  Port=2
  ki : Inport  Port=3
  i_max : Inport  Port=4
  Constant1 : Constant  Value=simIn.param.dt
  Data Type Conversion1 : DataTypeConversion  OutDataTypeStr=single
  IC1 : InitialCondition  Value=simIn.init.PIDP.I
  Integrator : MATLAB Function  TreatAsAtomicUnit=on
  Unit Delay1 : UnitDelay  InitialCondition=single(0)  SampleTime=-1  HasFrameUpgradeWarning=on
  integrator : Outport
  wires:
  i_max/1 -> Integrator/5(i_max)
  ki/1 -> Integrator/4(ki)
  Unit Delay1/1 -> Integrator/2(integrator)
  IC1/1 -> [integrator_out]
  [integrator_out] -> Unit Delay1/1
  limit_flg/1 -> Integrator/3(limit_flg)
  Constant1/1 -> Data Type Conversion1/1
  [integrator_out] -> integrator/1
  Integrator/1(integrator_out) -> IC1/1
  e/1 -> Integrator/1(error)
  Data Type Conversion1/1 -> Integrator/6(dt)
